simulink model "chaine_P6"  (R2023b)
settings: Solver=FixedStepDiscrete  StartTime=0.0  StopTime=10.0  RelTol=1e-3
values from neighbouring files (symbols this model uses):
  D7 = %d\n', F.rrc{3})    [partie6_chaine.m]
  decal6 = 0    [partie6_chaine.m]
undefined symbols (not defined in the file or in its folder): graine, graine_bruit, h6, L, nErrMax, sigma2, tab_b1, tab_b2, tab_I, tab_Q, Tb, Te_s
libraries: simulink x4
settings Model: Creator=e2405714  LastModifiedBy=e2405714

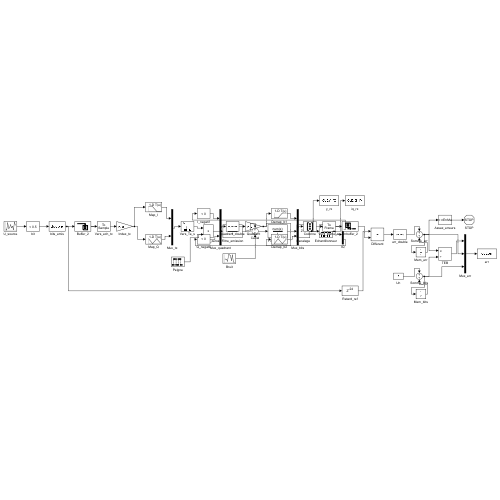
[thumbnail: Simulink's stored preview of the top-level diagram]
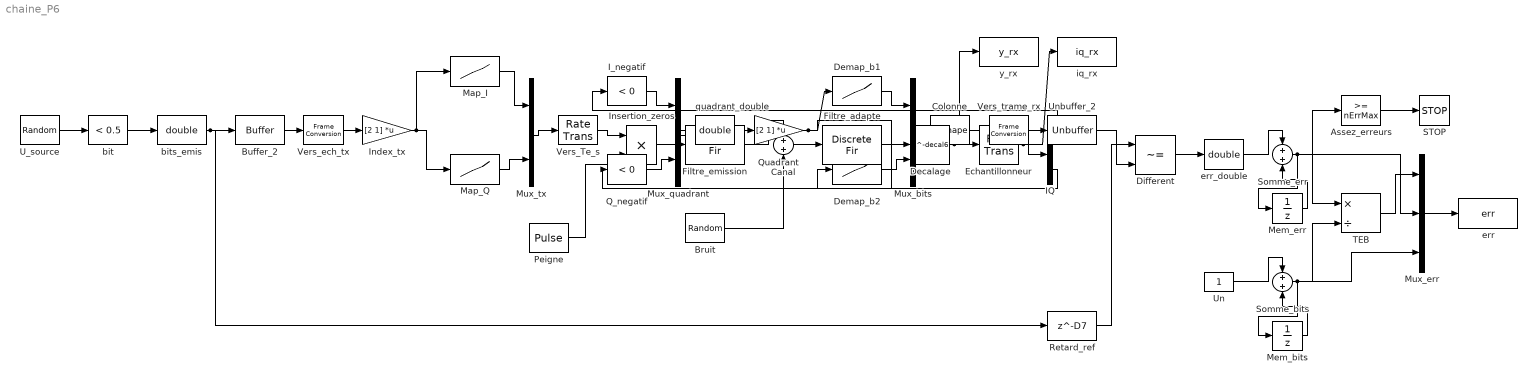
== system chaine_P6 ==
  Assez_erreurs : simulink/Logic and Bit Operations/Compare To Constant  relop=>=  const=nErrMax  OutDataTypeStr=boolean
  Bruit : RandomNumber  Mean=[0 0]  Variance=[sigma2 sigma2]  Seed=[graine_bruit graine_bruit+1]  SampleTime=Te_s
  Buffer_2 : Buffer  N=2
  Canal : Sum
  Colonne : Reshape  OutputDimensionality=Column vector (2-D)
  Decalage : Delay  DelayLength=decal6
  Demap_b1 : Lookup_n-D  NumberOfTableDimensions=1  BreakpointsForDimension1=0:3  Table=tab_b1  InternalRulePriority=Speed  RndMeth=Simplest
  Demap_b2 : Lookup_n-D  NumberOfTableDimensions=1  BreakpointsForDimension1=0:3  Table=tab_b2  InternalRulePriority=Speed  RndMeth=Simplest
  Different : RelationalOperator  Operator=~=  OutDataTypeStr=boolean  RndMeth=Simplest  InputSameDT=off
  Echantillonneur : RateTransition  OutPortSampleTime=Ts
  Filtre_adapte : DiscreteFir  Coefficients=fliplr(h6)
  Filtre_emission : DiscreteFir  Coefficients=h6
  IQ : Demux  Outputs=2
  I_negatif : simulink/Logic and Bit Operations/Compare To Constant  relop=<  const=0  OutDataTypeStr=boolean
  Index_tx : Gain  Gain=[2 1]  Multiplication=Matrix(K*u)
  Insertion_zeros : Product
  Map_I : Lookup_n-D  NumberOfTableDimensions=1  BreakpointsForDimension1=0:3  Table=tab_I  InternalRulePriority=Speed  RndMeth=Simplest
  Map_Q : Lookup_n-D  NumberOfTableDimensions=1  BreakpointsForDimension1=0:3  Table=tab_Q  InternalRulePriority=Speed  RndMeth=Simplest
  Mem_bits : UnitDelay  SampleTime=Tb  HasFrameUpgradeWarning=on
  Mem_err : UnitDelay  SampleTime=Tb  HasFrameUpgradeWarning=on
  Mux_bits : Mux  Inputs=2
  Mux_err : Mux  Inputs=3
  Mux_quadrant : Mux  Inputs=2
  Mux_tx : Mux  Inputs=2
  Peigne : DiscretePulseGenerator  Period=L  SampleTime=Te_s
  Q_negatif : simulink/Logic and Bit Operations/Compare To Constant  relop=<  const=0  OutDataTypeStr=boolean
  Quadrant : Gain  Gain=[2 1]  Multiplication=Matrix(K*u)
  Retard_ref : Delay  DelayLength=D7  SampleTime=Tb
  STOP : Stop
  Somme_bits : Sum
  Somme_err : Sum
  TEB : Product  Inputs=*/
  U_source : UniformRandomNumber  Minimum=0  Seed=graine  SampleTime=Tb
  Un : Constant  SampleTime=Tb
  Unbuffer_2 : Unbuffer
  Vers_Te_s : RateTransition  OutPortSampleTime=Te_s
  Vers_ech_tx : FrameConversion  OutFrame=Sample-based
  Vers_trame_rx : FrameConversion
  bit : simulink/Logic and Bit Operations/Compare To Constant  relop=<  const=0.5  OutDataTypeStr=boolean
  bits_emis : DataTypeConversion  OutDataTypeStr=double  SaturateOnIntegerOverflow=off  RndMeth=Floor
  err : ToWorkspace  VariableName=err  SampleTime=-1
  err_double : DataTypeConversion  OutDataTypeStr=double  SaturateOnIntegerOverflow=off  RndMeth=Floor
  iq_rx : ToWorkspace  VariableName=iq_rx  SampleTime=-1
      settings: MaxDataPoints=20000
  quadrant_double : DataTypeConversion  OutDataTypeStr=double  SaturateOnIntegerOverflow=off  RndMeth=Floor
  y_rx : ToWorkspace  VariableName=y_rx  SampleTime=-1
      settings: MaxDataPoints=20000
  wires:
  U_source/1 -> bit/1
  bit/1 -> bits_emis/1
  bits_emis/1 -> Buffer_2/1, Retard_ref/1
  Buffer_2/1 -> Vers_ech_tx/1
  Vers_ech_tx/1 -> Index_tx/1
  Index_tx/1 -> Map_I/1, Map_Q/1
  Map_I/1 -> Mux_tx/1
  Map_Q/1 -> Mux_tx/2
  Mux_tx/1 -> Vers_Te_s/1
  Vers_Te_s/1 -> Insertion_zeros/1
  Peigne/1 -> Insertion_zeros/2
  Insertion_zeros/1 -> Filtre_emission/1
  Filtre_emission/1 -> Canal/1
  Bruit/1 -> Canal/2
  Canal/1 -> Filtre_adapte/1
  Filtre_adapte/1 -> Decalage/1
  Decalage/1 -> Echantillonneur/1, y_rx/1
  Echantillonneur/1 -> iq_rx/1, IQ/1
  IQ/1 -> I_negatif/1
  IQ/2 -> Q_negatif/1
  I_negatif/1 -> Mux_quadrant/1
  Q_negatif/1 -> Mux_quadrant/2
  Mux_quadrant/1 -> quadrant_double/1
  quadrant_double/1 -> Quadrant/1
  Quadrant/1 -> Demap_b1/1, Demap_b2/1
  Demap_b1/1 -> Mux_bits/1
  Demap_b2/1 -> Mux_bits/2
  Mux_bits/1 -> Colonne/1
  Colonne/1 -> Vers_trame_rx/1
  Vers_trame_rx/1 -> Unbuffer_2/1
  Retard_ref/1 -> Different/1
  Unbuffer_2/1 -> Different/2
  Different/1 -> err_double/1
  err_double/1 -> Somme_err/1
  Mem_err/1 -> Somme_err/2
  Somme_err/1 -> Mem_err/1, TEB/1, Mux_err/2, Assez_erreurs/1
  Un/1 -> Somme_bits/1
  Mem_bits/1 -> Somme_bits/2
  Somme_bits/1 -> Mem_bits/1, TEB/2, Mux_err/3
  TEB/1 -> Mux_err/1
  Mux_err/1 -> err/1
  Assez_erreurs/1 -> STOP/1
